simulink model "sim_DP2_2026_SFC_Linear"  (R2025b)
settings: Solver=VariableStepAuto  StartTime=0.0  StopTime=Tsim  RelTol=1e-3
InitFcn:
  | myfile = 'sim_DP2_2026_SFC.p';
  | if exist(myfile, 'file')
  |     sim_DP2_2026_SFC
  | end
values from neighbouring files (symbols this model uses):
  A = [1 0 0 0 2.70127656662e-05 1.00008362958 0.0539210392304 0.167052905048 0.000996918625491 -3.04176177404e-06 0.993845368835 -0.00607175725634 ... (16 elements, 4x4)]    [Q2_Nonlinear_Workspace.mat]    (also in dp2_q1.m = sys_dt.A; dp2_q2_results.mat)
  Ac = [0 0 0 0 0 0 54.2357794574 167.674898301 1 0 -6.17904784847 -6.10719845489 ... (16 elements, 4x4)]    [Q2_Nonlinear_Workspace.mat]    (also in dp2_q1.m = [0, 0, 1, 0; dp2_q2_results.mat)
  B = [9.00986698557e-06 8.89404027496e-06 0.0179959975588 0.0177536761881]    [Q2_Nonlinear_Workspace.mat]    (also in dp2_q1.m = sys_dt.B; dp2_q2_results.mat)
  Bc = [0 0 18.0673913698 17.8573054236]    [Q2_Nonlinear_Workspace.mat]    (also in dp2_q1.m = [0; 0; b*kv/Delta0; c*kv/Delta0]; dp2_q2_results.mat)
  C = [1  0  0  0; 0  1  0  0]    [Q2_Nonlinear_Workspace.mat]    (also in dp2_q1.m = sys_dt.C; dp2_q2_results.mat)
  Cc = [1  0  0  0; 0  1  0  0]    [Q2_Nonlinear_Workspace.mat]    (also in dp2_q1.m = [1 0 0 0; dp2_q2_results.mat)
  F = [-0.145177182245 15.3825401153 -0.458881050593 0.765291685949]    [Q2_Nonlinear_Workspace.mat]    (also in dp2_q2.m = place(A,B,pz); dp2_q2_results.mat; main_SFC.m = place(A,B,pz))
  Lo = [0  0; 0  0; 0  0; 0  0]    [Q2_Nonlinear_Workspace.mat]    (also in main_SFC.m = place(A',C',po_z)')
  run_observer = 0    [Q2_Nonlinear_Workspace.mat]    (also in main_SFC.m = batch_case(2))
  ts = 0.001    [Q2_Nonlinear_Workspace.mat]    (also in dp2_q1.m; dp2_q2_results.mat)
  x_hat_o = [0 0 0 0]    [Q2_Nonlinear_Workspace.mat]    (also in main_SFC.m = [3*pi/180 -1*pi/180 0 0]')
settings Model: Creator=ricardoaguilera  LastModifiedBy=elinakim
settings SolverCC: AutoInsertRateTranBlk=on
settings DataIOCC: ReturnWorkspaceOutputs=off
settings DebuggingCC: AlgebraicLoopMsg=none

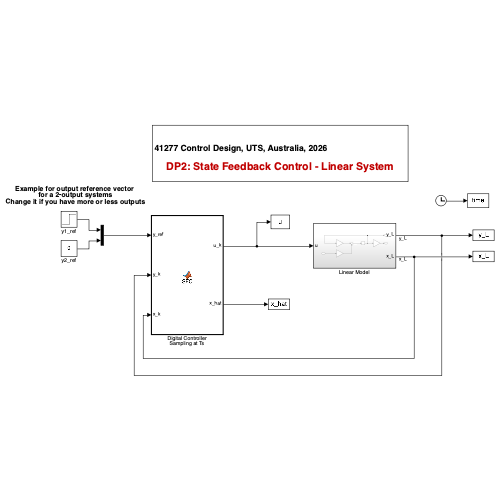
[thumbnail: Simulink's stored preview of the top-level diagram]
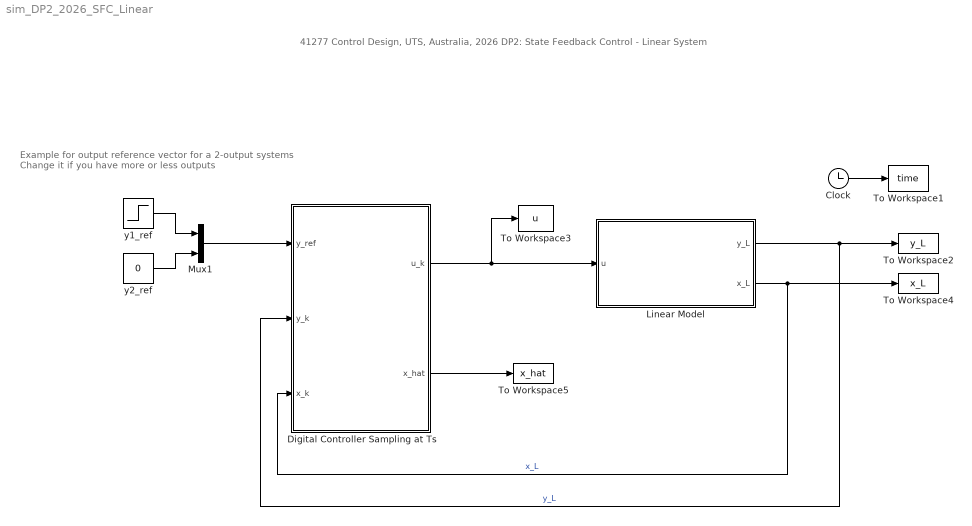
== system sim_DP2_2026_SFC_Linear ==
  note: Example for output reference vector
      | for a 2-output systems
      | Change it if you have more or less outputs
  note: 41277 Control Design, UTS, Australia, 2026
      |
      | DP2: State Feedback Control - Linear System
  Clock : Clock
  Digital Controller Sampling at Ts : MATLAB Function  TreatAsAtomicUnit=on  SystemSampleTime=ts
  Linear Model : Subsystem
  Mux1 : Mux  Inputs=2
  To Workspace1 : ToWorkspace  VariableName=time  SampleTime=ts
  To Workspace2 : ToWorkspace  VariableName=y_L  SampleTime=ts
  To Workspace3 : ToWorkspace  VariableName=u  SampleTime=ts
  To Workspace4 : ToWorkspace  VariableName=x_L  SampleTime=ts
  To Workspace5 : ToWorkspace  VariableName=x_hat  SampleTime=ts
  y1_ref : Step  After=5*pi/180  SampleTime=0
  y2_ref : Constant  Value=0
  wires:
  y1_ref/1 -> Mux1/1
  y2_ref/1 -> Mux1/2
  Clock/1 -> To Workspace1/1
  Mux1/1 -> Digital Controller Sampling at Ts/1(y_ref)
  Linear Model/2(x_L) -> Digital Controller Sampling at Ts/3(x_k), To Workspace4/1  "x_L"
  Linear Model/1(y_L) -> Digital Controller Sampling at Ts/2(y_k), To Workspace2/1  "y_L"
  Digital Controller Sampling at Ts/1(u_k) -> Linear Model/1(u), To Workspace3/1
  Digital Controller Sampling at Ts/2(x_hat) -> To Workspace5/1

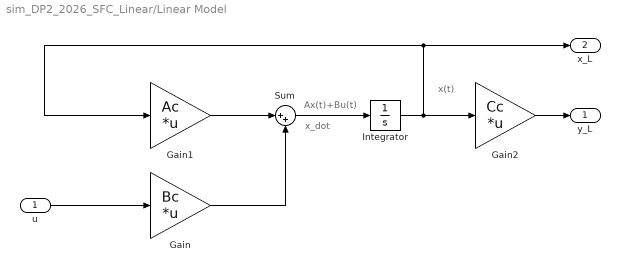
== system sim_DP2_2026_SFC_Linear/Linear Model ==
  note: x_dot
  note: Ax(t)+Bu(t)
  note: x(t)
  u : Inport
  Gain : Gain  Gain=Bc  Multiplication=Matrix(K*u)
  Gain1 : Gain  Gain=Ac  Multiplication=Matrix(K*u)
  Gain2 : Gain  Gain=Cc  Multiplication=Matrix(K*u)
  Integrator : Integrator
  Sum : Sum  Inputs=|++
  y_L : Outport  VectorParamsAs1DForOutWhenUnconnected=off
  x_L : Outport  Port=2  VectorParamsAs1DForOutWhenUnconnected=off
  wires:
  u/1 -> Gain/1
  Gain1/1 -> Sum/1
  Gain/1 -> Sum/2
  Sum/1 -> Integrator/1
  Integrator/1 -> Gain2/1, x_L/1, Gain1/1
  Gain2/1 -> y_L/1

== matlab function sim_DP2_2026_SFC_Linear/Digital Controller Sampling at Ts ==
  data: y_ref input; y_k input; x_k input; u_k output; F parameter; x_hat output; run_observer parameter; Lo parameter; A parameter; B parameter; C parameter; x_hat_o parameter
function [u_k, x_hat] = SFC(y_ref,y_k,x_k,F, ...
    run_observer,Lo,A,B,C,x_hat_o)

persistent x_hat_k

if isempty(x_hat_k)
    x_hat_k = x_hat_o;
end

x_hat = x_hat_k;

%% System size
m = size(B,2);

%% State references
x_ref = [y_ref(1); 0; 0; 0];
u_ref = 0;

u_k = zeros(m,1); % DO NOT DELETE

%% State-feedback control
if run_observer == 0
    u_k = -F*(x_k-x_ref) + u_ref;
else
    u_k = -F*(x_hat_k-x_ref) + u_ref;
end

%% Saturation: one motor, -10 V to +10 V
if u_k(1) > 10
    u_k(1) = 10;
elseif u_k(1) < -10
    u_k(1) = -10;
end

%% State-estimate update
y_hat = C*x_hat_k;
x_hat_k = A*x_hat_k + B*u_k + Lo*(y_k-y_hat);

end
